simulink model "Sistema_Control_04"  (R2026a)
settings: Solver=VariableStepAuto
values from neighbouring files (symbols this model uses):
  A = [-1/(C1*R1), 0, 0 ... (first row only)    [ControlDesign.m]    (also in fullObsCompensatorSim.m = sys.A; fundPro.m = sys_i.A; plotOFOLfullorder.m = sys_ol.A; plotOFOLreducedorder.m = sys_ol.A)
  B = [1/(C1*R1); 0; 0]    [ControlDesign.m]    (also in fullObsCompensatorSim.m = sys.B; fundPro.m = sys_i.B; plotOFOLfullorder.m = sys_ol.B; plotOFOLreducedorder.m = sys_ol.B)
  C = [0, 0, 1]    [ControlDesign.m]    (also in fullObsCompensatorSim.m = sys.C; fundPro.m = sys_i.C; plotOFOLfullorder.m = sys_ol.C; plotOFOLreducedorder.m = sys_ol.C)
  L = place(A', C', p_obs)'    [fullObsCompensatorSim.m]    (also in plotOFOLfullorder.m = place(A', C', eigenvalues)')
  P = [0 0 1;  1 0 0;  0 1 0]    [plotOFOLreducedorder.m]    (also in redObsCompensatorSim.m = [C; Nc'])
undefined symbols (not defined in the file or in its folder): AP, AQ, LC, Q
settings Model: Creator=Lorenzo  LastModifiedBy=Lorenzo

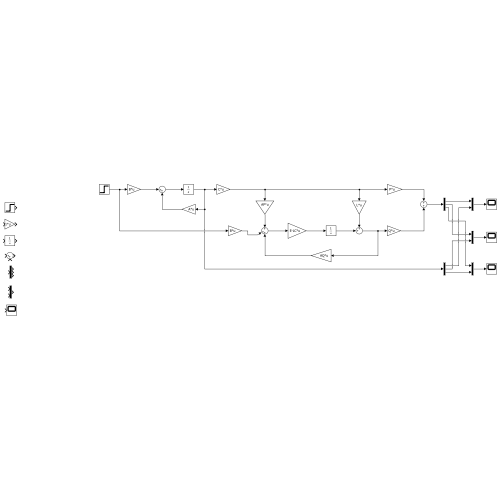
[thumbnail: Simulink's stored preview of the top-level diagram]
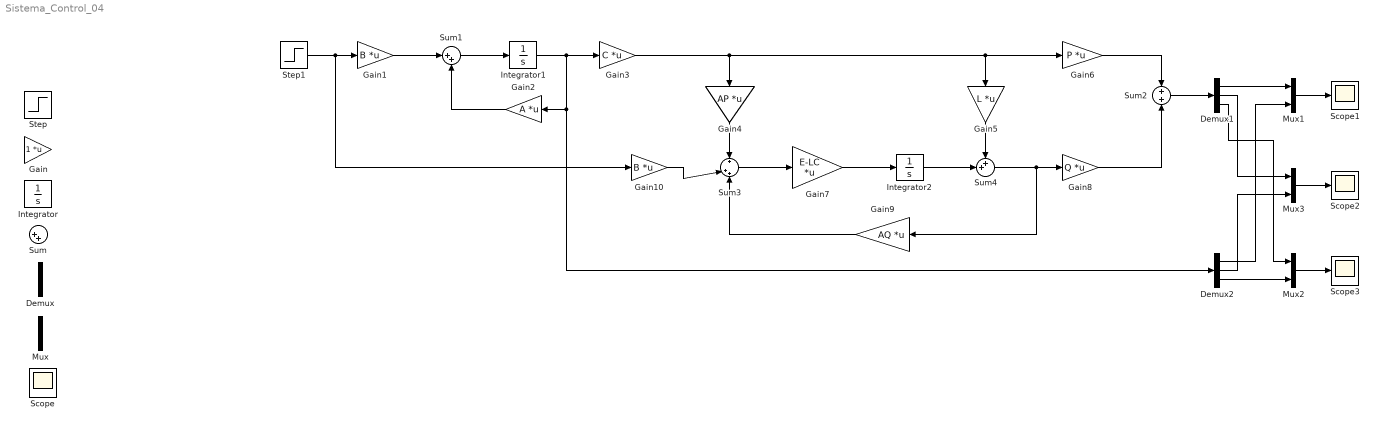
== system Sistema_Control_04 ==
  Demux : Demux  Outputs=3
  Demux1 : Demux  Outputs=3
  Demux2 : Demux  Outputs=3
  Gain : Gain  Multiplication=Matrix(K*u)
  Gain1 : Gain  Gain=B  Multiplication=Matrix(K*u)
  Gain10 : Gain  Gain=B  Multiplication=Matrix(K*u)
  Gain2 : Gain  Gain=A  Multiplication=Matrix(K*u)
  Gain3 : Gain  Gain=C  Multiplication=Matrix(K*u)
  Gain4 : Gain  Gain=AP  Multiplication=Matrix(K*u)
  Gain5 : Gain  Gain=L  Multiplication=Matrix(K*u)
  Gain6 : Gain  Gain=P  Multiplication=Matrix(K*u)
  Gain7 : Gain  Gain=E-LC  Multiplication=Matrix(K*u)
  Gain8 : Gain  Gain=Q  Multiplication=Matrix(K*u)
  Gain9 : Gain  Gain=AQ  Multiplication=Matrix(K*u)
  Integrator : Integrator
  Integrator1 : Integrator
  Integrator2 : Integrator
  Mux{,1..3} (4 alike) : Mux  Inputs=2
  Scope{,1..3} (4 alike) : Scope
      Scope2 settings: DataLoggingVariableName=ScopeData2
      Scope3 settings: DataLoggingVariableName=ScopeData3
  Step : Step  SampleTime=0
  Step1 : Step  SampleTime=0
  Sum : Sum  Inputs=|++
  Sum1 : Sum  Inputs=|++
  Sum2 : Sum  Inputs=+|+
  Sum3 : Sum  Inputs=+|++
  Sum4 : Sum  Inputs=++|
  wires:
  Step1/1 -> Gain10/1, Gain1/1
  Gain1/1 -> Sum1/1
  Sum1/1 -> Integrator1/1
  Integrator1/1 -> Demux2/1, Gain2/1, Gain3/1
  Gain2/1 -> Sum1/2
  Gain4/1 -> Sum3/1
  Sum3/1 -> Gain7/1
  Gain7/1 -> Integrator2/1
  Integrator2/1 -> Sum4/2
  Gain5/1 -> Sum4/1
  Sum4/1 -> Gain9/1, Gain8/1
  Gain8/1 -> Sum2/2
  Gain6/1 -> Sum2/1
  Gain9/1 -> Sum3/3
  Gain10/1 -> Sum3/2
  Gain3/1 -> Gain4/1, Gain6/1, Gain5/1
  Sum2/1 -> Demux1/1
  Demux1/1 -> Mux1/1
  Demux2/1 -> Mux1/2
  Demux1/2 -> Mux3/1
  Demux2/2 -> Mux3/2
  Demux1/3 -> Mux2/1
  Demux2/3 -> Mux2/2
  Mux2/1 -> Scope3/1
  Mux3/1 -> Scope2/1
  Mux1/1 -> Scope1/1
